simulink model "FOCwithLOAD"  (R2024b)
settings: Solver=FixedStepDiscrete  StartTime=0.0  StopTime=inf  RelTol=1e-3
PreLoadFcn:
  | % 自动加载同目录下的 linear_data.m，确保换机/首次打开可直接更新与编译
  | if ~evalin('base', 'exist(''Ts'',''var'') && exist(''pmsm'',''var'') && exist(''SMRC_I_Vsat_thresh'',''var'')')
  |     mdlDir_ = '';
  |     if bdIsLoaded('FOCwithLOAD'), mdlDir_ = fileparts(get_param('FOCwithLOAD', 'FileName')); end
  |     if isempty(mdlDir_), mdlDir_ = fileparts(which('FOCwithLOAD')); end
  |     if isempty(mdlDir_), mdlDir_ = pwd; end
  |     dataFile_ = fullfile(mdlDir_, 'linear_data.m');
  |     if isfile(dataFile_)
  |         assignin('base', 'linearDataFileTmp_', dataFile_);
  |         evalin('base', 'run(linearDataFileTmp_); clear linearDataFileTmp_');
  |     end
  |     clear mdlDir_ dataFile_
  | end
InitFcn:
  | % 自动加载同目录下的 linear_data.m，确保换机/首次打开可直接更新与编译
  | if ~evalin('base', 'exist(''Ts'',''var'') && exist(''pmsm'',''var'') && exist(''SMRC_I_Vsat_thresh'',''var'')')
  |     mdlDir_ = '';
  |     if bdIsLoaded('FOCwithLOAD'), mdlDir_ = fileparts(get_param('FOCwithLOAD', 'FileName')); end
  |     if isempty(mdlDir_), mdlDir_ = fileparts(which('FOCwithLOAD')); end
  |     if isempty(mdlDir_), mdlDir_ = pwd; end
  |     dataFile_ = fullfile(mdlDir_, 'linear_data.m');
  |     if isfile(dataFile_)
  |         assignin('base', 'linearDataFileTmp_', dataFile_);
  |         evalin('base', 'run(linearDataFileTmp_); clear linearDataFileTmp_');
  |     end
  |     clear mdlDir_ dataFile_
  | end
values from neighbouring files (symbols this model uses):
  a_hat = Kt_eff / (pmsm.J * omega_pu_base)    [linear_data.m]
  ADRC_B0 = 6055    [linear_data.m]
  ADRC_Wc = 3.2e-3    (= 0.0032)    [linear_data.m]
  ADRC_Wo = 30    [linear_data.m]
  alpha_ppc = exp(-lambda_ppc*Ts_speed)    [linear_data.m]
  b_hat = pmsm.B/pmsm.J    [linear_data.m]
  beta1 = single(2.0 * w_o)    [linear_data.m]
  beta2_sat_scale = 0.2    [linear_data.m]
  dataType = 'single'    [linear_data.m]
  gamma_reset = 0.9    [linear_data.m]
  inv_a_hat = 1/double(a_hat)    [linear_data.m]
  k_xi = 55    [linear_data.m]
  Kff = 0.98931745    [linear_data.m]
  lambda_ppc = 45    [linear_data.m]
  P_inf_const = 0.004    [linear_data.m]
  PI_params = mcb_SetControllerParameters(pmsm,inverter,PU_System,T_pwm,Ts,Ts_speed)    [linear_data.m]
  pmsm2 = pmsm    [linear_data.m]
  s_limit_sat = 0.9    [linear_data.m]
  speedRPM2mmps = pmlsm.mmps_per_rpm    [linear_data.m]
  target = mcb_SetProcessorDetails('F28379D',PWM_frequency)    [linear_data.m]
  Ts = T_pwm    (= 5e-05)    [linear_data.m]
  Ts_motor = T_pwm/2    (= 2.5e-05)    [linear_data.m]
  Ts_speed = 1*Ts    (= 5e-05)    [linear_data.m]
  w_o = single(200.0)    [linear_data.m]
  z2_limit = single(100.0)    [linear_data.m]
undefined symbols (not defined in the file or in its folder): DiscIntNeverNeededParam, Down, GPTRIP1SEL, GPTRIP2SEL, innerPI, inverter, inverter2, outerPI, pmlsm, pmsm, Tctr, TZ1, TZ2, Up
libraries: c2802xlib x13, simulink x10, c2837xDlib x6, c280xlib x6, slpidlib x5, svdschedulerlib x4, mcbcontrolslib x4, mcbpositiondecoderlib x2, mcbpmsmnonlinearlib x2, autolibpmsmexterior x2, mcbplantlib x2, svdutilitieslib x1
(part 5 of 5)

== system FOCwithLOAD/Motor2 Torque control/Control_System/Closed Loop Control1/Controller/Filter1 ==
  R(n) : Inport
  Gain : Gain  Gain=1/(Tctr*innerPI.Filter.w0+1)
  Gain1 : Gain  Gain=(Tctr*innerPI.Filter.w0)/(Tctr*innerPI.Filter.w0+1)
  Sum : Sum  Inputs=|++
  Unit Delay : UnitDelay  SampleTime=-1  HasFrameUpgradeWarning=on
  Y(n) : Outport
  wires:
  Unit Delay/1 -> Gain/1  "Y(n-1)"
  Sum/1 -> Y(n)/1, Unit Delay/1  "Y(n)"
  Gain/1 -> Sum/2
  R(n)/1 -> Gain1/1
  Gain1/1 -> Sum/1

== system FOCwithLOAD/Motor2 Torque control/Control_System/Closed Loop Control1/Controller/Inner D axis Controller ==
  iD_req : Inport
  iD_fdbk : Inport  Port=2
  Constant1 : Constant  Value=innerPI.iD.Discrete.Kp  OutDataTypeStr=single
  Constant2 : Constant  Value=innerPI.iD.Discrete.KiTctr  OutDataTypeStr=single
  Constant6 : Constant  Value=0  OutDataTypeStr=single
  Discrete PI Controller with anti-windup & reset : slpidlib/PID Controller  Controller=PI  Form=Parallel  TimeDomain=Discrete-time  UseExternalTs=off  SampleTime=-1  IntegratorMethod=Forward Euler  FilterMethod=Forward Euler  ControllerParametersSource=external  P=1  I=1  UseKiTs=on  D=0  UseExternalDerivativeSource=off  N=100  UseFilter=on  TunerSelectOption=Transfer Function Based (PID Tuner App)  InitialConditionSource=external  InitialConditionForIntegrator=0  InitialConditionForFilter=0  DifferentiatorICPrevScaledInput=0  ExternalReset=none  TrackingMode=off  Kt=1  LimitOutput=on  SatLimitsSource=internal  UpperSaturationLimit=0.8*inverter.V_dc*sqrt(3)/3  LowerSaturationLimit=-0.8*inverter.V_dc*sqrt(3)/3  LinearizeAsGain=on  AntiWindupMode=clamping  Kb=1  LimitIntegrator=off  UpperIntegratorSaturationLimit=inf  LowerIntegratorSaturationLimit=-inf  RndMeth=Simplest  POutMin=[]  POutMax=[]  IOutMin=[]  IOutMax=[]  DOutMin=[]  DOutMax=[]  NOutMin=[]  NOutMax=[]  SumOutMin=[]  SumOutMax=[]  SaturationOutDataTypeStr=Inherit: Inherit via back propagation  SaturationOutMin=[]  SaturationOutMax=[]  PParamMin=[]  PParamMax=[]  IParamMin=[]  IParamMax=[]  DParamMin=[]  DParamMax=[]  NParamMin=[]  NParamMax=[]  KbParamMin=[]  KbParamMax=[]  KtParamMin=[]  KtParamMax=[]  KbOutMin=[]  KbOutMax=[]  KtOutMin=[]  KtOutMax=[]  IntegratorOutMin=[]  IntegratorOutMax=[]  FilterOutMin=[]  FilterOutMax=[]  SumI1OutMin=[]  SumI1OutMax=[]  SumI2OutMin=[]  SumI2OutMax=[]  SumI3OutMin=[]  SumI3OutMax=[]  SumI4OutMin=[]  SumI4OutMax=[]  SumDOutMin=[]  SumDOutMax=[]  DifferentiatorOutMin=[]  DifferentiatorOutMax=[]  FilterDiffOutCoefMin=[]  FilterDiffOutCoefMax=[]  ReciprocalOutMin=[]  ReciprocalOutMax=[]  SumDenOutMin=[]  SumDenOutMax=[]  SumNumOutMin=[]  SumNumOutMax=[]  DivideOutMin=[]  DivideOutMax=[]  UdiffTsProdOutMin=[]  UdiffTsProdOutMax=[]  NTsProdOutMin=[]  NTsProdOutMax=[]  UintegralTsProdOutMin=[]  UintegralTsProdOutMax=[]  UngainTsProdOutMin=[]  UngainTsProdOutMax=[]  ClampingZeroOutDataTypeStr=Inherit: Inherit via back propagation  ClampingZeroOutMin=[]  ClampingZeroOutMax=[]  FilterDenConstantOutDataTypeStr=Inherit: Inherit via back propagation  FilterDenConstantOutMin=[]  FilterDenConstantOutMax=[]  PCopyOutDataTypeStr=Inherit: Inherit via back propagation  PCopyOutMin=[]  PCopyOutMax=[]  NCopyOutDataTypeStr=Inherit: Inherit via back propagation  NCopyOutMin=[]  NCopyOutMax=[]  IntegratorContinuousStateAttributes=''  IntegratorStateMustResolveToSignalObject=off  IntegratorRTWStateStorageClass=Auto  FilterContinuousStateAttributes=''  FilterStateMustResolveToSignalObject=off  FilterRTWStateStorageClass=Auto  ParallelPVariant=ExternalParameters  IdealPVariant=Disabled  IVariant=ExternalParameters  DVariant=Disabled  IntegratorVariant=Discrete  SatVariant=Enabled  AWVariant=DiscClampingParallel  PCopyVariant=Disabled  TRVariant=Disabled  FdbkBlocksVariant=Forward  IdealPFdbkVariant=Disabled  SatFdbkVariant=Disabled  DerivativeFilterVariant=Disabled  NVariant=Disabled  NCopyVariant=Disabled_SignalSpec  FilterICVariant=Disabled  IntegratorICVariant=ExternalICs  ExternalResetVariant=Disabled  TRSumVariant=Passthrough  SumFdbkVariant=Disabled  SumVariant=Sum_PI  TsampFilterVariant=InternalTs  TsampNgainVariant=Passthrough  TsampIntegralVariant=Disabled_SignalSpec  ExternalSaturationOutDataTypeStr=Inherit: Same as second input  DerivativeSourceVariant=Disabled  PreIntVariant=InternalPreInt
      settings: LibrarySourceBlock=mcbcontrolslib/PI Controller
  Sum1 : Sum  Inputs=|+-
  uD_req : Outport
  wires:
  Constant6/1 -> Discrete PI Controller with anti-windup & reset/4
  Discrete PI Controller with anti-windup & reset/1 -> uD_req/1
  Constant2/1 -> Discrete PI Controller with anti-windup & reset/3
  Constant1/1 -> Discrete PI Controller with anti-windup & reset/2
  iD_fdbk/1 -> Sum1/2
  iD_req/1 -> Sum1/1
  Sum1/1 -> Discrete PI Controller with anti-windup & reset/1

== system FOCwithLOAD/Motor2 Torque control/Control_System/Closed Loop Control1/Controller/Inner Q axis Controller ==
  iQ_req : Inport
  iQ_fdbk : Inport  Port=2
  Constant1 : Constant  Value=innerPI.iQ.Discrete.KiTctr  OutDataTypeStr=single
  Constant2 : Constant  Value=innerPI.iQ.Discrete.Kp  OutDataTypeStr=single
  Constant6 : Constant  Value=0  OutDataTypeStr=single
  Discrete PI Controller with anti-windup & reset : slpidlib/PID Controller  Controller=PI  Form=Parallel  TimeDomain=Discrete-time  UseExternalTs=off  SampleTime=-1  IntegratorMethod=Forward Euler  FilterMethod=Forward Euler  ControllerParametersSource=external  P=1  I=1  UseKiTs=on  D=0  UseExternalDerivativeSource=off  N=100  UseFilter=on  TunerSelectOption=Transfer Function Based (PID Tuner App)  InitialConditionSource=external  InitialConditionForIntegrator=0  InitialConditionForFilter=0  DifferentiatorICPrevScaledInput=0  ExternalReset=none  TrackingMode=off  Kt=1  LimitOutput=on  SatLimitsSource=internal  UpperSaturationLimit=0.8*inverter.V_dc*sqrt(3)/3  LowerSaturationLimit=-0.8*inverter.V_dc*sqrt(3)/3  LinearizeAsGain=on  AntiWindupMode=clamping  Kb=1  LimitIntegrator=off  UpperIntegratorSaturationLimit=inf  LowerIntegratorSaturationLimit=-inf  RndMeth=Simplest  POutMin=[]  POutMax=[]  IOutMin=[]  IOutMax=[]  DOutMin=[]  DOutMax=[]  NOutMin=[]  NOutMax=[]  SumOutMin=[]  SumOutMax=[]  SaturationOutDataTypeStr=Inherit: Inherit via back propagation  SaturationOutMin=[]  SaturationOutMax=[]  PParamMin=[]  PParamMax=[]  IParamMin=[]  IParamMax=[]  DParamMin=[]  DParamMax=[]  NParamMin=[]  NParamMax=[]  KbParamMin=[]  KbParamMax=[]  KtParamMin=[]  KtParamMax=[]  KbOutMin=[]  KbOutMax=[]  KtOutMin=[]  KtOutMax=[]  IntegratorOutMin=[]  IntegratorOutMax=[]  FilterOutMin=[]  FilterOutMax=[]  SumI1OutMin=[]  SumI1OutMax=[]  SumI2OutMin=[]  SumI2OutMax=[]  SumI3OutMin=[]  SumI3OutMax=[]  SumI4OutMin=[]  SumI4OutMax=[]  SumDOutMin=[]  SumDOutMax=[]  DifferentiatorOutMin=[]  DifferentiatorOutMax=[]  FilterDiffOutCoefMin=[]  FilterDiffOutCoefMax=[]  ReciprocalOutMin=[]  ReciprocalOutMax=[]  SumDenOutMin=[]  SumDenOutMax=[]  SumNumOutMin=[]  SumNumOutMax=[]  DivideOutMin=[]  DivideOutMax=[]  UdiffTsProdOutMin=[]  UdiffTsProdOutMax=[]  NTsProdOutMin=[]  NTsProdOutMax=[]  UintegralTsProdOutMin=[]  UintegralTsProdOutMax=[]  UngainTsProdOutMin=[]  UngainTsProdOutMax=[]  ClampingZeroOutDataTypeStr=Inherit: Inherit via back propagation  ClampingZeroOutMin=[]  ClampingZeroOutMax=[]  FilterDenConstantOutDataTypeStr=Inherit: Inherit via back propagation  FilterDenConstantOutMin=[]  FilterDenConstantOutMax=[]  PCopyOutDataTypeStr=Inherit: Inherit via back propagation  PCopyOutMin=[]  PCopyOutMax=[]  NCopyOutDataTypeStr=Inherit: Inherit via back propagation  NCopyOutMin=[]  NCopyOutMax=[]  IntegratorContinuousStateAttributes=''  IntegratorStateMustResolveToSignalObject=off  IntegratorRTWStateStorageClass=Auto  FilterContinuousStateAttributes=''  FilterStateMustResolveToSignalObject=off  FilterRTWStateStorageClass=Auto  ParallelPVariant=ExternalParameters  IdealPVariant=Disabled  IVariant=ExternalParameters  DVariant=Disabled  IntegratorVariant=Discrete  SatVariant=Enabled  AWVariant=DiscClampingParallel  PCopyVariant=Disabled  TRVariant=Disabled  FdbkBlocksVariant=Forward  IdealPFdbkVariant=Disabled  SatFdbkVariant=Disabled  DerivativeFilterVariant=Disabled  NVariant=Disabled  NCopyVariant=Disabled_SignalSpec  FilterICVariant=Disabled  IntegratorICVariant=ExternalICs  ExternalResetVariant=Disabled  TRSumVariant=Passthrough  SumFdbkVariant=Disabled  SumVariant=Sum_PI  TsampFilterVariant=InternalTs  TsampNgainVariant=Passthrough  TsampIntegralVariant=Disabled_SignalSpec  ExternalSaturationOutDataTypeStr=Inherit: Same as second input  DerivativeSourceVariant=Disabled  PreIntVariant=InternalPreInt
      settings: LibrarySourceBlock=mcbcontrolslib/PI Controller
  Sum : Sum  Inputs=|+-
  uQ_req : Outport
  wires:
  iQ_fdbk/1 -> Sum/2
  iQ_req/1 -> Sum/1
  Constant2/1 -> Discrete PI Controller with anti-windup & reset/2
  Constant1/1 -> Discrete PI Controller with anti-windup & reset/3
  Constant6/1 -> Discrete PI Controller with anti-windup & reset/4
  Discrete PI Controller with anti-windup & reset/1 -> uQ_req/1
  Sum/1 -> Discrete PI Controller with anti-windup & reset/1

== system FOCwithLOAD/Motor2 Torque control/Control_System/Closed Loop Control1/SVPWM/InvClark ==
  note: $i_a=i_\alpha\\ i_b=-\frac{1}{2}i_\alpha+\frac{\sqrt{3}}{2}i_\beta\\ i_c=-\frac{1}{2}i_\alpha-\frac{\sqrt{3}}{2}i_\beta$
  note: u_c_spwm
  note: u_b_spwm
  note: u_a_spwm
  u_alpha : Inport
  u_beta : Inport  Port=2
  Gain : Gain  Gain=-1/2
  Gain1 : Gain  Gain=sqrt(3)/2
  Mux : Mux  Inputs=3
  Sum : Sum  Inputs=|++
  Sum1 : Sum  Inputs=-+|
  u_abc_spwm : Outport
  wires:
  Mux/1 -> u_abc_spwm/1
  Sum1/1 -> Mux/3
  Sum/1 -> Mux/2
  u_alpha/1 -> Gain/1, Mux/1
  Gain1/1 -> Sum/2, Sum1/1
  u_beta/1 -> Gain1/1
  Gain/1 -> Sum/1, Sum1/2

== system FOCwithLOAD/Motor2 Torque control/Control_System/Closed Loop Control1/SVPWM/ei_t ==
  note: $e_i(t)=\frac{1}{2}(1-u^\ast_{max})+\frac{1}{2}(-1-u^\ast_{min})=-\frac{1}{2}(u^\ast_{max}+u^*_{min})$
  u_abc_spwm : Inport
  Demux : Demux  Outputs=3
  Gain : Gain  Gain=-1/2
  Max : MinMax  Function=max  Inputs=3
  Min : MinMax  Inputs=3
  Sum : Sum  Inputs=|++
  sit : Outport
  wires:
  Gain/1 -> sit/1
  Sum/1 -> Gain/1
  Max/1 -> Sum/2
  Min/1 -> Sum/1
  Demux/3 -> Min/3, Max/3
  Demux/2 -> Min/2, Max/2
  Demux/1 -> Min/1, Max/1
  u_abc_spwm/1 -> Demux/1

== system FOCwithLOAD/Motor2 Torque control/Control_System/Closed Loop Control1/Sample Choice/AB 采样计算2 ==
  Iabc : Inport
  AB : ActionPort  ActionPortLabel=else
  Demux : Demux  Outputs=3
  Mux : Mux  Inputs=3
  Sum : Sum  Inputs=--
  Terminator : Terminator
  IABC : Outport
  wires:
  Iabc/1 -> Demux/1
  Mux/1 -> IABC/1
  Demux/2 -> Sum/2, Mux/2
  Demux/1 -> Sum/1, Mux/1
  Sum/1 -> Mux/3
  Demux/3 -> Terminator/1

== system FOCwithLOAD/Motor2 Torque control/Control_System/Closed Loop Control1/Sample Choice/AC 采样计算1 ==
  Iabc : Inport
  AC : ActionPort  ActionPortLabel=elseif(u2 >= u1 & u2 >= u3)
  Demux : Demux  Outputs=3
  Mux : Mux  Inputs=3
  Sum : Sum  Inputs=|--
  Terminator : Terminator
  IABC : Outport
  wires:
  Demux/3 -> Mux/3, Sum/2
  Demux/1 -> Mux/1, Sum/1
  Iabc/1 -> Demux/1
  Mux/1 -> IABC/1
  Sum/1 -> Mux/2
  Demux/2 -> Terminator/1

== system FOCwithLOAD/Motor2 Torque control/Control_System/Closed Loop Control1/Sample Choice/BC 采样计算 ==
  Iabc : Inport
  选择BC : ActionPort  ActionPortLabel=if(u1 >= u2 & u1 >= u3)
  Demux : Demux  Outputs=3
  Mux : Mux  Inputs=3
  Sum : Sum  Inputs=|--
  Terminator : Terminator
  IABC : Outport
  wires:
  Iabc/1 -> Demux/1
  Demux/1 -> Terminator/1
  Mux/1 -> IABC/1
  Demux/2 -> Sum/1, Mux/2
  Demux/3 -> Mux/3, Sum/2
  Sum/1 -> Mux/1

== system FOCwithLOAD/Motor2 Torque control/Input Scaling/Calculate Phase Currents/Data_Type/Data_Type_Fixed_Point ==
  In1 : Inport
  Data Type Conversion : DataTypeConversion  OutDataTypeStr=fixdt(1,32,17)  ConvertRealWorld=Stored Integer (SI)  RndMeth=Simplest  SaturateOnIntegerOverflow=off
  Data Type Conversion1 : DataTypeConversion  OutDataTypeStr=dataType  RndMeth=Simplest  SaturateOnIntegerOverflow=off
  Q17 per unit conversion : ArithShift  BitShiftNumber=-6
  Iabc_meas_Real : Outport
  wires:
  In1/1 -> Q17 per unit conversion/1
  Data Type Conversion1/1 -> Iabc_meas_Real/1
  Data Type Conversion/1 -> Data Type Conversion1/1
  Q17 per unit conversion/1 -> Data Type Conversion/1

== system FOCwithLOAD/Motor2 Torque control/Input Scaling/Calculate Phase Currents/Data_Type/Data_Type_Float ==
  In1 : Inport
  Get ADC Voltage : Gain  Gain=target.ADC_Vref /target.ADC_MaxCount  OutDataTypeStr=dataType  RndMeth=Simplest
  Get Currents : Gain  Gain=1/inverter2.ISenseVoltPerAmp  RndMeth=Simplest  OutDataTypeStr=Inherit: Same as input
  Iabc_meas_Real : Outport
  wires:
  Get ADC Voltage/1 -> Get Currents/1
  In1/1 -> Get ADC Voltage/1
  Get Currents/1 -> Iabc_meas_Real/1

== matlab function FOCwithLOAD/Motor1 Speed control/Input Scaling/ Calculate Position and Speed/Pos2Ang ==
  data: cnt input; theta_pu output
function theta_pu = Pos2Ang(cnt)
c0 = cnt(1);
K  = uint32(20000);
r  = mod(c0, K);
if bitand(c0, uint32(2147483648)) ~= uint32(0)
    r = mod(r + uint32(12704), K);
end
theta_pu = single(r) * single(0.00005);
end

== matlab function FOCwithLOAD/Motor2 Torque control/Input Scaling/ Calculate Position and Speed/AlignFSM2 ==
  data: AlignMode2 output; EnMtr2TrqCtrl output; EnMtr2Ctrl output; Cmd input; PosOffset2 output; PosRaw input; EnRun input; Ts input; AlignTheta2 output
function [AlignMode2, EnMtr2TrqCtrl, EnMtr2Ctrl, PosOffset2, AlignTheta2] = AlignFSM2(Cmd, PosRaw, EnRun, Ts) %#codegen
% 电机2 两段式校准状态机：
%   Cmd==2: 0~0.50s 预定位至 90deg (0.25 PU) 脱离180deg死点；>=0.50s 拉回 0deg (0 PU)；
%           >=1.10s 锁存零点并置位 calValid2=1
%   Cmd==0 且 calValid2==1 且 EnRun~=0: 转矩闭环运行；其它停机
persistent off2 calValid2 tAlign2
if isempty(calValid2)
    off2 = single(0);
    calValid2 = uint8(0);
    tAlign2 = single(0);
end
T_PRE   = single(0.50);
T_LATCH = single(1.10);
AlignMode2 = false;
EnMtr2TrqCtrl = false;
AlignTheta2 = single(0);
if Cmd == 2
    AlignMode2 = true;
    if tAlign2 < T_PRE
        AlignTheta2 = single(0.25);
        calValid2 = uint8(0);
    else
        AlignTheta2 = single(0);
        if tAlign2 >= T_LATCH
            off2 = single(PosRaw(1));
            calValid2 = uint8(1);
        end
    end
    if tAlign2 < single(10.0)
        tAlign2 = tAlign2 + single(Ts(1));
    end
else
    tAlign2 = single(0);
    if (Cmd == 0) && (calValid2 == uint8(1)) && (EnRun ~= 0)
        EnMtr2TrqCtrl = true;
    end
end
EnMtr2Ctrl = EnMtr2TrqCtrl || AlignMode2;
PosOffset2 = off2;
end

== matlab function FOCwithLOAD/Motor2 Torque control/Input Scaling/ Calculate Position and Speed/Pos2Ang ==
  data: cnt input; theta_pu output
function theta_pu = Pos2Ang(cnt)
c0 = cnt(1);
K  = uint32(20000);
r  = mod(c0, K);
if bitand(c0, uint32(2147483648)) ~= uint32(0)
    r = mod(r + uint32(12704), K);
end
theta_pu = single(r) * single(0.00005);
end

== matlab function FOCwithLOAD/Motor1 Speed control/Outer Controller/ppc/MATLAB Function ==
  data: SpeedPU_req input; g_eso output; SpeedPU_fdbk input; Iq_ref_prev input
function g_eso = g_eso_ctrl(SpeedPU_req, SpeedPU_fdbk, Iq_ref_prev)
%#codegen

%% 固定参数
enable_eso = true;

Ts_speed = single(5e-5);

p_inf    = single(0.006);
iq_max_A = single(8.0);   
% q 轴电流上限，单位 A

iq_min_A = single(-8.0);  
% q 轴电流下限，单位 A

e_ss_on = single(0.02);  
% 稳态误差判据，单位 PU
% abs(e) < e_ss_on 才允许认为误差足够小

dw_ss_on = single(0.20);  
% 稳态速度变化率判据，单位 PU/s
% dw_filt < dw_ss_on 才允许认为速度变化足够慢

T_steady_on = single(0.02);  
% 满足稳态条件后，需要持续这么长时间才允许 ESO 接入，单位 s

N_steady_on = int32(T_steady_on / Ts_speed);  
% 稳态持续时间对应的采样点数

tau_dw = single(0.005);  
% 速度变化率低通滤波时间常数，单位 s

alpha_dw = Ts_speed / (tau_dw + Ts_speed);  
% 速度变化率一阶低通滤波系数

tau_eso_gate = single(0.01);  
% ESO 接入平滑时间常数，单位 s
% 越大接入越慢

alpha_gate = Ts_speed / (tau_eso_gate + Ts_speed);  
% g_eso 平滑接入的一阶滤波系数

%% 持久化状态
persistent req_prev speed_fdbk_prev dw_filt steady_cnt eso_enable_latch g_eso_state initialized

if isempty(initialized)
    initialized       = true;
    req_prev          = single(SpeedPU_req);
    speed_fdbk_prev   = single(SpeedPU_fdbk);
    dw_filt           = single(0.0);
    steady_cnt        = int32(0);
    eso_enable_latch  = false;
    g_eso_state       = single(0.0);
end

%% 1) 误差
e = single(SpeedPU_req - SpeedPU_fdbk);

%% 2) ref_jump
ref_jump = abs(single(SpeedPU_req - req_prev)) > p_inf;

%% 3) is_sat
is_sat_hi = Iq_ref_prev > (iq_max_A - single(0.05));
is_sat_lo = Iq_ref_prev < (iq_min_A + single(0.05));
is_sat = is_sat_hi || is_sat_lo;

%% 4) dw_raw / dw_filt
dw_raw = abs(single((SpeedPU_fdbk - speed_fdbk_prev) / Ts_speed));
dw_filt = dw_filt + alpha_dw * (dw_raw - dw_filt);
dw_filt = single(dw_filt);

%% 5) steady_candidate
steady_candidate = (abs(e) < e_ss_on) && ...
                   (dw_filt < dw_ss_on) && ...
                   (~is_sat);

%% 6) steady_cnt / eso_enable_latch
if ref_jump
    steady_cnt = int32(0);
    eso_enable_latch = false;
else
    if ~eso_enable_latch
        if steady_candidate
            if steady_cnt < N_steady_on
                steady_cnt = steady_cnt + 1;
            end
            if steady_cnt >= N_steady_on
                eso_enable_latch = true;
            end
        else
            steady_cnt = int32(0);
        end
    end
end

%% 7) g_eso_cmd
if enable_eso && eso_enable_latch
    g_eso_cmd = single(1.0);
else
    g_eso_cmd = single(0.0);
end

%% 8) g_eso 平滑接入
g_eso_state = g_eso_state + alpha_gate * (g_eso_cmd - g_eso_state);
g_eso_state = single(g_eso_state);

if g_eso_state > single(1.0)
    g_eso_state = single(1.0);
elseif g_eso_state < single(0.0)
    g_eso_state = single(0.0);
end

%% 9) 更新状态
req_prev        = single(SpeedPU_req);
speed_fdbk_prev = single(SpeedPU_fdbk);

%% 10) 输出
g_eso = single(g_eso_state);
end

== matlab function FOCwithLOAD/Motor1 Speed control/Outer Controller/MATLAB Function ==
  data: SpeedPU_req input; Iq_ref_A output; SpeedPU_fdbk input; e_out output; P_out output; s_out output; xi_out output; edot_des_out output; iq_ff_A_out output; iq_fb_A_out output; iq_unsat_A_out output; iq_eso_A_out output; z1_out output; z2_out output; g_eso_out output
function [Iq_ref_A, e_out, P_out, s_out, xi_out, edot_des_out, ...
          iq_ff_A_out, iq_fb_A_out, iq_unsat_A_out, ...
          iq_eso_A_out, z1_out, z2_out, g_eso_out] = ...
          PPC_ESO_SpeedLoop_WithFF_Fixed(SpeedPU_req, SpeedPU_fdbk)
%#codegen
%
% PPC + ESO speed loop (fixed)
%
% 修复点：
% 1) 保留原始 PPC + friction feedforward 结构
% 2) ESO 观测器模型改为： y_dot = -b_hat*y + a_hat*iq + d
%    避免把已知阻尼项重复当成扰动补偿
% 3) 启动阶段仍然由原始 PPC 主导
% 4) 稳态后 ESO 平滑接入
%
% Inputs:
%   SpeedPU_req   : speed reference (PU), base = 3000 rpm
%   SpeedPU_fdbk  : speed feedback  (PU), base = 3000 rpm
%
% Outputs:
%   Iq_ref_A        : q-axis current reference (A)
%   e_out           : speed error
%   P_out           : performance bound
%   s_out           : normalized error
%   xi_out          : transformed error
%   edot_des_out    : desired error derivative
%   iq_ff_A_out     : friction feedforward current (A)
%   iq_fb_A_out     : PPC feedback current (A)
%   iq_unsat_A_out  : current command before saturation (A)
%   iq_eso_A_out    : ESO compensation current (A)
%   z1_out          : ESO observed speed (PU)
%   z2_out          : ESO observed lumped disturbance (PU/s)
%   g_eso_out       : ESO blending factor [0,1]

%% =========================
% 0) 调试开关
% =========================
enable_eso = true;   % 先设 false 可验证其行为应与原始纯PPC一致

%% =========================
% 1) Fixed parameters
% =========================
Ts_speed = single(5e-5);   % 与你原始PPC一致：0.5 ms

% Motor parameters
J  = single(2.6450e-05);   % kg*m^2
B  = single(3.1136e-04);   % kg*m^2/s
p  = single(3.0);          % pole pairs
Ke = single(11.9557);      % Vpk_LL/krpm

% Speed PU base = 3000 rpm
N_pu_base_rpm = single(3000.0);
omega_pu_base = single(2.0*pi) * N_pu_base_rpm / single(60.0);  % rad/s

%% =========================
% 2) Motor constants
% =========================
FluxPM = Ke / (single(sqrt(3.0)) * single(2.0*pi) * single(1000.0) * p / single(60.0));
Kt_eff = single(1.5) * p * FluxPM;   % ~0.0989 Nm/A

% Speed model in PU:
%   wdot_pu = a_hat * iq_A - b_hat * w_pu + d
a_hat = Kt_eff / (J * omega_pu_base);   % pu/s per A
b_hat = B / J;                          % 1/s

%% =========================
% 3) PPC parameters
% 完全沿用你原始代码
% =========================
p_inf       = single(0.006);
eps_p       = single(1e-3);
s0_star     = single(0.8);
s_limit     = single(0.9);

lambda_ppc  = single(35.0);
k_xi        = single(55.0);
gamma_reset = single(0.9);

% Current saturation
iq_max_A = single(8.0);
iq_min_A = single(-8.0);

one  = single(1.0);
half = single(0.5);

%% =========================
% 4) ESO parameters
% =========================
w_o      = single(150.0);
beta1    = single(2.0 * w_o);
beta2    = single(w_o * w_o);
z2_limit = single(100.0);

beta2_sat_scale = single(0.2);

% ESO接入时间常数
tau_eso_gate = single(0.02);   % 20 ms
alpha_gate = Ts_speed / (tau_eso_gate + Ts_speed);

%% =========================
% 5) Steady-state detection parameters
% =========================
e_ss_on     = single(0.006);   % 约18 rpm
dw_ss_on    = single(0.20);    % PU/s
T_steady_on = single(0.02);    % 连续20ms满足稳态
N_steady_on = int32(T_steady_on / Ts_speed);

tau_dw   = single(0.005);      % 5 ms
alpha_dw = Ts_speed / (tau_dw + Ts_speed);

%% =========================
% 6) Persistent states
% =========================
persistent Pk_prev req_prev initialized
persistent z1 z2 iq_ref_prev
persistent speed_fdbk_prev dw_filt steady_cnt eso_enable_latch g_eso

if isempty(initialized)
    initialized = true;

    % 原始PPC初始化
    req_prev = single(SpeedPU_req);
    e0 = single(SpeedPU_req - SpeedPU_fdbk);
    P0 = max(abs(e0) / s0_star, p_inf + eps_p);
    Pk_prev = single(P0);

    % ESO初始化
    z1 = single(SpeedPU_fdbk);
    z2 = single(0.0);
    iq_ref_prev = single(0.0);

    % 稳态检测初始化
    speed_fdbk_prev = single(SpeedPU_fdbk);
    dw_filt = single(0.0);
    steady_cnt = int32(0);
    eso_enable_latch = false;
    g_eso = single(0.0);
end

%% =========================
% 7) Speed error
% =========================
e = single(SpeedPU_req - SpeedPU_fdbk);

%% =========================
% 8) Performance bound P(k)
% 完全沿用原始PPC
% =========================
ref_jump    = abs(single(SpeedPU_req - req_prev)) > p_inf;
err_trigger = abs(e) > gamma_reset * Pk_prev;

if ref_jump || err_trigger
    Pk = max(abs(e) / s0_star, p_inf + eps_p);
else
    alpha = exp(-lambda_ppc * Ts_speed);
    Pk = p_inf + alpha * (Pk_prev - p_inf);
end
Pk = single(Pk);

%% =========================
% 9) Normalized error
% =========================
den = max(Pk, p_inf + eps_p);
s = e / den;
s = single(s);

if s > s_limit
    s_sat = s_limit;
elseif s < -s_limit
    s_sat = -s_limit;
else
    s_sat = s;
end
s_sat = single(s_sat);

%% =========================
% 10) Transformed error
% =========================
xi = half * log((one + s_sat) / (one - s_sat));
xi = single(xi);

%% =========================
% 11) Desired error derivative
% 完全沿用原始PPC
% =========================
Pdot = -lambda_ppc * (Pk - p_inf);
Pdot = single(Pdot);

term1 = (Pdot / den) * e;
term1 = single(term1);

term2 = Pk * (one - s_sat * s_sat) * k_xi * xi;
term2 = single(term2);

edot_des = term1 - term2;
edot_des = single(edot_des);

%% =========================
% 12) 原始PPC电流分解
% =========================
% friction feedforward
omega_mech = single(SpeedPU_fdbk) * omega_pu_base;
iq_ff_A = (B * omega_mech) / Kt_eff;
iq_ff_A = single(iq_ff_A);

% PPC feedback current
iq_fb_A = (-edot_des) / a_hat;
iq_fb_A = single(iq_fb_A);

%% =========================
% 13) LESO 后台持续观测（修复后的模型）
% 正确模型：
%   y_dot = -b_hat*y + a_hat*iq + d
% Observer:
%   z1_dot = -b_hat*z1 + z2 + a_hat*u - beta1*(z1-y)
%   z2_dot = -beta2*(z1-y)
% =========================
err_obs = single(z1 - SpeedPU_fdbk);

is_sat_hi = iq_ref_prev > (iq_max_A - single(0.05));
is_sat_lo = iq_ref_prev < (iq_min_A + single(0.05));
is_sat = is_sat_hi || is_sat_lo;

z1_next = z1 + Ts_speed * ( -b_hat * z1 + z2 + a_hat * iq_ref_prev - beta1 * err_obs );
z1_next = single(z1_next);

if is_sat
    beta2_eff = beta2_sat_scale * beta2;
else
    beta2_eff = beta2;
end

z2_next = z2 + Ts_speed * ( -beta2_eff * err_obs );
z2_next = single(z2_next);

if z2_next > z2_limit
    z2_next = z2_limit;
elseif z2_next < -z2_limit
    z2_next = -z2_limit;
end
z2_next = single(z2_next);

%% =========================
% 14) Steady-state detection
% =========================
dw_raw = abs(single((SpeedPU_fdbk - speed_fdbk_prev) / Ts_speed));
dw_filt = dw_filt + alpha_dw * (dw_raw - dw_filt);
dw_filt = single(dw_filt);

steady_candidate = (abs(e) < e_ss_on) && ...
                   (dw_filt < dw_ss_on) && ...
                   (~is_sat);

% 新指令来了，重新回到纯PPC
if ref_jump
    steady_cnt = int32(0);
    eso_enable_latch = false;
end

if ~eso_enable_latch
    if steady_candidate
        if steady_cnt < N_steady_on
            steady_cnt = steady_cnt + 1;
        end
        if steady_cnt >= N_steady_on
            eso_enable_latch = true;
        end
    else
        steady_cnt = int32(0);
    end
end

%% =========================
% 15) ESO blending factor
% =========================
if enable_eso && eso_enable_latch
    g_eso_cmd = single(1.0);
else
    g_eso_cmd = single(0.0);
end

g_eso = g_eso + alpha_gate * (g_eso_cmd - g_eso);
g_eso = single(g_eso);

%% =========================
% 16) ESO compensation current
% 只补未知扰动，不再重复补已知阻尼项
% =========================
iq_eso_A = -g_eso * z2_next / a_hat;
iq_eso_A = single(iq_eso_A);

%% =========================
% 17) Total current command
% 关键：保持原始结构 iq_ff + iq_fb，再加 ESO 未知扰动补偿
% =========================
iq_unsat_A = iq_ff_A + iq_fb_A + iq_eso_A;
iq_unsat_A = single(iq_unsat_A);

if iq_unsat_A > iq_max_A
    Iq_ref_A = iq_max_A;
elseif iq_unsat_A < iq_min_A
    Iq_ref_A = iq_min_A;
else
    Iq_ref_A = iq_unsat_A;
end
Iq_ref_A = single(Iq_ref_A);

%% =========================
% 18) Update states
% =========================
Pk_prev         = single(Pk);
req_prev        = single(SpeedPU_req);

z1              = single(z1_next);
z2              = single(z2_next);
iq_ref_prev     = single(Iq_ref_A);

speed_fdbk_prev = single(SpeedPU_fdbk);

%% =========================
% 19) Outputs
% =========================
e_out          = single(e);
P_out          = single(Pk);
s_out          = single(s_sat);
xi_out         = single(xi);
edot_des_out   = single(edot_des);

iq_ff_A_out    = single(iq_ff_A);
iq_fb_A_out    = single(iq_fb_A);
iq_unsat_A_out = single(iq_unsat_A);

iq_eso_A_out   = single(iq_eso_A);
z1_out         = single(z1);
z2_out         = single(z2);
g_eso_out      = single(g_eso);

end

== matlab function FOCwithLOAD/Motor1 Speed control/Outer Controller/ESO+PPC ==
  data: SpeedPU_req input; Iq_ref_A output; SpeedPU_fdbk input; e_out output; P_out output; s_out output; xi_out output; edot_des_out output; iq_ff_A_out output; iq_fb_A_out output; iq_unsat_A_out output; iq_eso_A_out output; z1_out output; z2_out output; g_eso_out output; omega_o_dyn_out output
function [Iq_ref_A, e_out, P_out, s_out, xi_out, edot_des_out, ...
          iq_ff_A_out, iq_fb_A_out, iq_unsat_A_out, ...
          iq_eso_A_out, z1_out, z2_out, g_eso_out, omega_o_dyn_out] = ...
          PPC_ESO_SpeedLoop_WithFF_Fixed(SpeedPU_req, SpeedPU_fdbk)
%#codegen
%
% PPC + ESO speed loop (验证专用版：带omega_o_dyn_out，便于观察动态增益变化)

%% =========================
% 0) 调试开关
% =========================
enable_eso = true;

%% =========================
% 1) Fixed parameters
% =========================
Ts_speed = single(5e-5);
J = single(2.6450e-05); B = single(3.1136e-04); p = single(3.0); Ke = single(11.9557);
N_pu_base_rpm = single(3000.0);
omega_pu_base = single(2.0*pi) * N_pu_base_rpm / single(60.0);
FluxPM = Ke / (single(sqrt(3.0)) * single(2.0*pi) * single(1000.0) * p / single(60.0));
Kt_eff = single(1.5) * p * FluxPM;
a_hat = Kt_eff / (J * omega_pu_base);
b_hat = B / J;

%% =========================
% 3) PPC parameters
% =========================
p_inf = single(0.006); eps_p = single(1e-3); s0_star = single(0.8); s_limit = single(0.9);
lambda_ppc = single(35.0); k_xi = single(55.0); gamma_reset = single(0.9);
iq_max_A = single(8.0); iq_min_A = single(-8.0);
one = single(1.0); half = single(0.5);

%% =========================
% 4) ESO parameters（保守动态增益）
% =========================
w_o = single(150.0);
lambda_xi = single(2.5);                % 验证用值
omega_min = single(0.0);
omega_max = single(350.0);

%lambda_xi = single(0.0);
%omega_min = w_o;
%omega_max = w_o;

tau_gain = single(0.0015);
alpha_gain = Ts_speed / (tau_gain + Ts_speed);

beta2_sat_scale = single(0.2);
z2_limit = single(120.0);

tau_eso_gate = single(0.02);
alpha_gate = Ts_speed / (tau_eso_gate + Ts_speed);

%% =========================
% 5) Steady-state detection parameters
% =========================
e_ss_on = single(0.006); dw_ss_on = single(0.20);
T_steady_on = single(0.02); N_steady_on = int32(T_steady_on / Ts_speed);
tau_dw = single(0.005); alpha_dw = Ts_speed / (tau_dw + Ts_speed);

%% =========================
% 6) Persistent states
% =========================
persistent Pk_prev req_prev initialized
persistent z1 z2 iq_ref_prev
persistent speed_fdbk_prev dw_filt steady_cnt eso_enable_latch g_eso omega_o_dyn
if isempty(initialized)
    initialized = true;
    req_prev = single(SpeedPU_req);
    e0 = single(SpeedPU_req - SpeedPU_fdbk);
    P0 = max(abs(e0) / s0_star, p_inf + eps_p);
    Pk_prev = single(P0);
    z1 = single(SpeedPU_fdbk);
    z2 = single(0.0);
    iq_ref_prev = single(0.0);
    speed_fdbk_prev = single(SpeedPU_fdbk);
    dw_filt = single(0.0);
    steady_cnt = int32(0);
    eso_enable_latch = false;
    g_eso = single(0.0);
    omega_o_dyn = single(w_o);
end

%% =========================
% 7~12) 原PPC + FF（完全不变）
% =========================
e = single(SpeedPU_req - SpeedPU_fdbk);

ref_jump = abs(single(SpeedPU_req - req_prev)) > p_inf;
err_trigger = abs(e) > gamma_reset * Pk_prev;
if ref_jump || err_trigger
    Pk = max(abs(e) / s0_star, p_inf + eps_p);
else
    alpha = exp(-lambda_ppc * Ts_speed);
    Pk = p_inf + alpha * (Pk_prev - p_inf);
end
Pk = single(Pk);

den = max(Pk, p_inf + eps_p);
s = e / den;
if s > s_limit, s_sat = s_limit; elseif s < -s_limit, s_sat = -s_limit; else, s_sat = s; end
s_sat = single(s_sat);

xi = half * log((one + s_sat) / (one - s_sat));
xi = single(xi);

Pdot = -lambda_ppc * (Pk - p_inf);
term1 = (Pdot / den) * e;
term2 = Pk * (one - s_sat * s_sat) * k_xi * xi;
edot_des = term1 - term2; edot_des = single(edot_des);

omega_mech = single(SpeedPU_fdbk) * omega_pu_base;
iq_ff_A = (B * omega_mech) / Kt_eff; iq_ff_A = single(iq_ff_A);
iq_fb_A = (-edot_des) / a_hat; iq_fb_A = single(iq_fb_A);

%% =========================
% 13) 动态增益 + LESO
% =========================
omega_dyn_cmd = w_o * (one + lambda_xi * abs(xi));
if omega_dyn_cmd > omega_max
    omega_dyn_cmd = omega_max;
elseif omega_dyn_cmd < omega_min
    omega_dyn_cmd = omega_min;
end
omega_o_dyn = omega_o_dyn + alpha_gain * (omega_dyn_cmd - omega_o_dyn);
omega_o_dyn = single(omega_o_dyn);

beta1 = single(2.0 * omega_o_dyn);
beta2 = single(omega_o_dyn * omega_o_dyn);

err_obs = single(z1 - SpeedPU_fdbk);
is_sat_hi = iq_ref_prev > (iq_max_A - single(0.05));
is_sat_lo = iq_ref_prev < (iq_min_A + single(0.05));
is_sat = is_sat_hi || is_sat_lo;

z1_next = z1 + Ts_speed * (-b_hat * z1 + z2 + a_hat * iq_ref_prev - beta1 * err_obs);
z1_next = single(z1_next);

if is_sat
    beta2_eff = beta2_sat_scale * beta2;
else
    beta2_eff = beta2;
end
beta2_eff = single(beta2_eff);

z2_next = z2 + Ts_speed * (-beta2_eff * err_obs);
z2_next = single(z2_next);
if z2_next > z2_limit, z2_next = z2_limit; elseif z2_next < -z2_limit, z2_next = -z2_limit; end
z2_next = single(z2_next);

%% =========================
% 14) Steady-state detection（不变）
% =========================
dw_raw = abs(single((SpeedPU_fdbk - speed_fdbk_prev) / Ts_speed));
dw_filt = dw_filt + alpha_dw * (dw_raw - dw_filt);
dw_filt = single(dw_filt);
steady_candidate = (abs(e) < e_ss_on) && (dw_filt < dw_ss_on) && (~is_sat);
if ref_jump
    steady_cnt = int32(0); eso_enable_latch = false;
end
if ~eso_enable_latch
    if steady_candidate
        if steady_cnt < N_steady_on, steady_cnt = steady_cnt + 1; end
        if steady_cnt >= N_steady_on, eso_enable_latch = true; end
    else
        steady_cnt = int32(0);
    end
end

%% =========================
% 15~19) blending + 补偿 + 输出（不变）
% =========================
if enable_eso && eso_enable_latch
    g_eso_cmd = single(1.0);
else
    g_eso_cmd = single(0.0);
end
g_eso = g_eso + alpha_gate * (g_eso_cmd - g_eso);
g_eso = single(g_eso);

iq_eso_A = -g_eso * z2_next / a_hat;
iq_eso_A = single(iq_eso_A);

iq_unsat_A = iq_ff_A + iq_fb_A + iq_eso_A;
Iq_ref_A = max(iq_min_A, min(iq_max_A, iq_unsat_A));
Iq_ref_A = single(Iq_ref_A);

Pk_prev = single(Pk); req_prev = single(SpeedPU_req);
z1 = single(z1_next); z2 = single(z2_next);
iq_ref_prev = single(Iq_ref_A); speed_fdbk_prev = single(SpeedPU_fdbk);

e_out = single(e); P_out = single(Pk); s_out = single(s_sat); xi_out = single(xi);
edot_des_out = single(edot_des);
iq_ff_A_out = single(iq_ff_A); iq_fb_A_out = single(iq_fb_A);
iq_unsat_A_out = single(iq_unsat_A); iq_eso_A_out = single(iq_eso_A);
z1_out = single(z1); z2_out = single(z2); g_eso_out = single(g_eso);
omega_o_dyn_out = single(omega_o_dyn);   % ← 新增，便于验证动态增益变化

end

== matlab function FOCwithLOAD/Motor1 Speed control/Input Scaling/ Calculate Position and Speed/AlignFSM ==
  data: Cmd input; AlignMode output; PosRaw input; Ts input; EnClosedLoop output; PosOffset output; EnRun input; AlignTheta output
function [AlignMode, EnClosedLoop, PosOffset, AlignTheta] = AlignFSM(Cmd, PosRaw, Ts, EnRun) %#codegen
% 电机1 两段式校准状态机：
%   Cmd==1: 0~0.50s 预定位至 90deg (0.25 PU) 脱离180deg死点；>=0.50s 拉回 0deg (0 PU)；
%           >=1.10s 锁存零点并置位 calValid=1
%   Cmd==0 且 calValid==1 且 EnRun~=0: 闭环运行；其它停机
persistent off calValid tAlign
if isempty(calValid)
    off = single(0);
    calValid = uint8(0);
    tAlign = single(0);
end
T_PRE   = single(0.50);
T_LATCH = single(1.10);
AlignMode = false;
EnClosedLoop = false;
AlignTheta = single(0);
if Cmd == 1
    AlignMode = true;
    if tAlign < T_PRE
        AlignTheta = single(0.25);
        calValid = uint8(0);
    else
        AlignTheta = single(0);
        if tAlign >= T_LATCH
            off = single(PosRaw(1));
            calValid = uint8(1);
        end
    end
    if tAlign < single(10.0)
        tAlign = tAlign + single(Ts(1));
    end
else
    tAlign = single(0);
    if (Cmd == 0) && (calValid == uint8(1)) && (EnRun ~= 0)
        EnClosedLoop = true;
    end
end
PosOffset = off;
end
